simulink model "W09_E1_LoopOnce"  (R2024b)
settings: Solver=ode45  StartTime=0.0  StopTime=t_end  MaxStep=0.02  RelTol=1e-3
PreLoadFcn:
  | % W09_E1_LoopOnce 기본 파라미터 (모델을 열 때 자동 실행)
  | defs = { 'K',2 ; 'w_in',1 ; 't_end',40 ;
  |          'numG',1 ; 'denG',[1 2 1 0] };
  | for ii = 1:size(defs,1)
  |     if ~evalin('base', sprintf('exist(''%s'',''var'')', defs{ii,1}))
  |         assignin('base', defs{ii,1}, defs{ii,2});
  |     end
  | end
  | clear defs ii
values from neighbouring files (symbols this model uses):
  K = 0.5    [W09_02_pm_to_time.m]    (also in W09_03_run_simulink.m; W09_07_examples.m)
  w_in = w_list(i)    [W09_07_examples.m]
undefined symbols (not defined in the file or in its folder): denG, numG
settings Model: Creator=admin  LastModifiedBy=admin

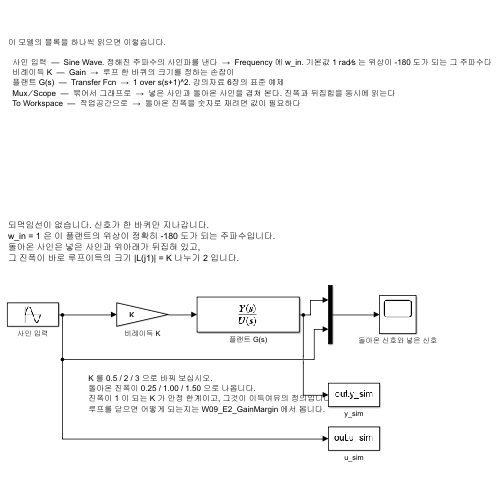
[thumbnail: Simulink's stored preview of the top-level diagram]
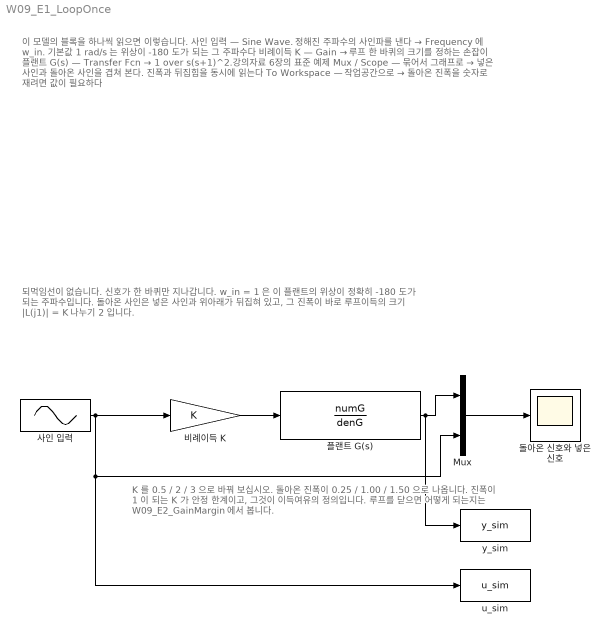
== system W09_E1_LoopOnce ==
  note: 되먹임선이 없습니다. 신호가 한 바퀴만 지나갑니다.
      | w_in = 1 은 이 플랜트의 위상이 정확히 -180 도가 되는 주파수입니다.
      | 돌아온 사인은 넣은 사인과 위아래가 뒤집혀 있고,
      | 그 진폭이 바로 루프이득의 크기 |L(j1)| = K 나누기 2 입니다.
  note: K 를 0.5 / 2 / 3 으로 바꿔 보십시오.
      | 돌아온 진폭이 0.25 / 1.00 / 1.50 으로 나옵니다.
      | 진폭이 1 이 되는 K 가 안정 한계이고, 그것이 이득여유의 정의입니다.
      | 루프를 닫으면 어떻게 되는지는 W09_E2_GainMargin 에서 봅니다.
  note: 이 모델의 블록을 하나씩 읽으면 이렇습니다.
      |
      |   사인 입력  —  Sine Wave. 정해진 주파수의 사인파를 낸다  →  Frequency 에 w_in. 기본값 1 rad∕s 는 위상이 -180 도가 되는 그 주파수다
      |   비례이득 K  —  Gain  →  루프 한 바퀴의 크기를 정하는 손잡이
      |   플랜트 G(s)  —  Transfer Fcn  →  1 over s(s+1)^2. 강의자료 6장의 표준 예제
      |   Mux ∕ Scope  —  묶어서 그래프로  →  넣은 사인과 돌아온 사인을 겹쳐 본다. 진폭과 뒤집힘을 동시에 읽는다
      |   To Workspace  —  작업공간으로  →  돌아온 진폭을 숫자로 재려면 값이 필요하다
  Mux : Mux  Inputs=2
  u_sim : ToWorkspace  VariableName=u_sim  SaveFormat=Timeseries  SampleTime=-1
  y_sim : ToWorkspace  VariableName=y_sim  SaveFormat=Timeseries  SampleTime=-1
  돌아온 신호와 넣은 신호 : Scope
  비례이득 K : Gain  Gain=K
  사인 입력 : Sin  Frequency=w_in  SampleTime=0
  플랜트 G(s) : TransferFcn  Numerator=numG  Denominator=denG
  wires:
  사인 입력/1 -> Mux/2, u_sim/1, 비례이득 K/1
  비례이득 K/1 -> 플랜트 G(s)/1
  플랜트 G(s)/1 -> Mux/1, y_sim/1
  Mux/1 -> 돌아온 신호와 넣은 신호/1
